simulink model "RETINA_X_Rural_DigitalTwin"  (R2026a)
settings: Solver=VariableStepAuto  StopTime=1
settings Model: Creator=anika  LastModifiedBy=anika

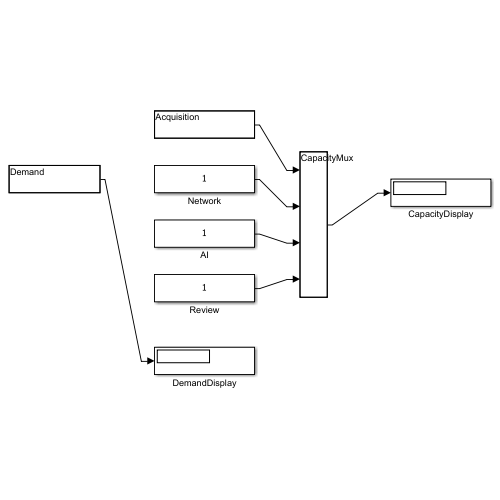
[thumbnail: Simulink's stored preview of the top-level diagram]
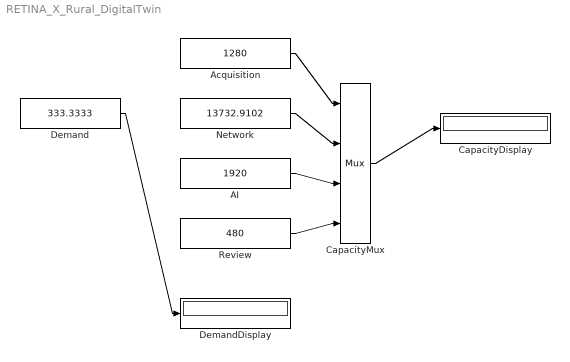
== system RETINA_X_Rural_DigitalTwin ==
  AI : Constant  Value=1920
  Acquisition : Constant  Value=1280
  CapacityDisplay : Display
  CapacityMux : Mux
  Demand : Constant  Value=333.3333
  DemandDisplay : Display
  Network : Constant  Value=13732.9102
  Review : Constant  Value=480
  wires:
  Acquisition/1 -> CapacityMux/1
  Network/1 -> CapacityMux/2
  AI/1 -> CapacityMux/3
  Review/1 -> CapacityMux/4
  CapacityMux/1 -> CapacityDisplay/1
  Demand/1 -> DemandDisplay/1
